simulink subsystem "SkewMatrix"  (R2024b)
settings: Solver=VariableStepAuto  StartTime=0.0  StopTime=10.0  RelTol=1e-3
settings Model: Creator=marco  LastModifiedBy=ferru

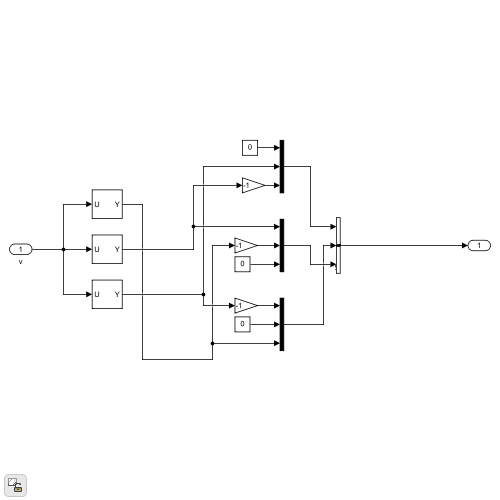
[thumbnail: Simulink's stored preview of the top-level diagram]
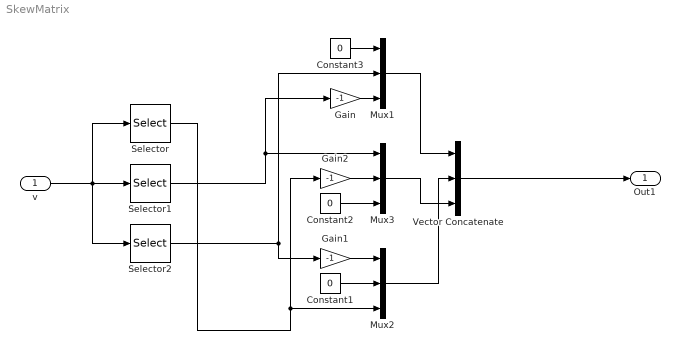
== system SkewMatrix ==
  v : Inport
  Constant1 : Constant  Value=0
  Constant2 : Constant  Value=0
  Constant3 : Constant  Value=0
  Gain : Gain  Gain=-1
  Gain1 : Gain  Gain=-1
  Gain2 : Gain  Gain=-1
  Mux1 : Mux  Inputs=3
  Mux2 : Mux  Inputs=3
  Mux3 : Mux  Inputs=3
  Selector : Selector  NumberOfDimensions=2  InputPortWidth=3  IndexOptions=Index vector (dialog),Select all  Indices=1,1  OutputSizes=1,1
  Selector1 : Selector  NumberOfDimensions=2  InputPortWidth=3  IndexOptions=Index vector (dialog),Select all  Indices=2,1  OutputSizes=1,1
  Selector2 : Selector  NumberOfDimensions=2  InputPortWidth=3  IndexOptions=Index vector (dialog),Select all  Indices=3,1  OutputSizes=1,1
  Vector Concatenate : Concatenate  NumInputs=3  Mode=Multidimensional array  ConcatenateDimension=2
  Out1 : Outport
  wires:
  Selector2/1 -> Gain1/1, Mux1/2
  Constant1/1 -> Mux2/2
  Mux2/1 -> Vector Concatenate/2
  Constant2/1 -> Mux3/3
  Selector1/1 -> Mux3/1, Gain/1
  Vector Concatenate/1 -> Out1/1
  Gain2/1 -> Mux3/2
  Mux1/1 -> Vector Concatenate/1
  Selector/1 -> Gain2/1, Mux2/3
  Mux3/1 -> Vector Concatenate/3
  Gain/1 -> Mux1/3
  Constant3/1 -> Mux1/1
  Gain1/1 -> Mux2/1
  v/1 -> Selector/1, Selector2/1, Selector1/1
